simulink model "ps_model"  (R2025b)
settings: Solver=ode23tb  StartTime=0.0  StopTime=simlength  FixedStep=tc  MaxStep=tc
values from neighbouring files (symbols this model uses):
  omega_grid_emulator_nom = w_grid    (= 314.159265359)    [grid_emulator.m]
  omega_grid_nom = w_grid    (= 314.159265359)    [grid_emulator.m]
  ugrid_factor = 1    [grid_emulator.m]
  V_phase_normalization_factor = Vgrid_phase_normalization_factor    [grid_emulator.m]
  Vdc_base = 720    [grid_emulator.m]
  vn_eta_pu = 0    [grid_emulator.m]
  vn_xi_pu = 0    [grid_emulator.m]
  vp_xi_pu = 1    [grid_emulator.m]
undefined symbols (not defined in the file or in its folder): CFi, fnom, fPWM_INV, i_nom, ki_i, ki_u, kp_i, kp_u, Ld2_trafo_out, magnitude, n10, number_of_cells, omega_nom, Q, q1Kalman, q2Kalman, q3Kalman, R_RLload, Rd2_trafo_out, rKalman, tc, time_load_step, ts_afe, ts_inv, tsample, u_nom, Vdc_nom
libraries: fl_lib x120, nesl_utility x67, ee_lib x7, cstblocks x4, moving_average_filter x4, single_phase_transformer_lib x3, lithium_ion_cell_lib x1, simulink x1, threephase_inductor_lib x1
(part 3 of 4)

== system ps_model/inverter/MOS based inverter/inverter ==
  Simulink-PS Converter{,1..5} (6 alike) : nesl_utility/Simulink-PS Converter  PhysicalDomain=network_engine_domain  SubClassName=ps_input  LeftPortType=input  RightPortType=output  PseudoPeriodic=off  Frequencies=[]  NoiseDistribution=none  NoiseParameters=[]  Unit=V  AffineConversion=on  FilteringAndDerivatives=provide  SimscapeFilterOrder=1  InputFilterTimeConstant=0.001  UdotUserProvided=0
  mosfet_1 : Subsystem
      settings: PortSchema="{\"entries\":[{\"content\":{\"sides\":[{\"content\":{\"connectorIds\":[\"LConn1\"]},\"type\":\"ConnectorPlacement.EquallySpacedRectSide\",\"uuid\":\"9277da8d-d460-43e6-8478-dd662f15d226\"},{\"content\":{\"connectorIds\":[],\"side\":\"RIGHT\"},\"type\":\"ConnectorPlacement.EquallySpacedRectSide\",\"uuid\":\"a7ece396-f1d9-4f4f-a05b-db1fc65d6e1d\"},{\"content\":{\"connectorIds\":[\"LConn2\"],\"side\":\"TOP\"},\"type\":\"ConnectorPlacement.EquallySpacedRectSide\",\"uuid\":\"fdd70777-e9cf-4317-afb6-cae87f75d5b0\"},{\"content\":{\"connectorIds\":[\"RConn1\"],\"side\":\"BOTTOM\"},\"type\":\"ConnectorPlacement.EquallySpacedRectSide\",\"uuid\":\"2353ed68-b1a1-4775-9ca9-31e268d5443b\"}]},\"type\":\"ConnectorPlacement.EquallySpacedConnector\",\"uuid\":\"d5479f4c-4e65-4791-adcb-73df11f88590\"}],\"packageUris\":[\"http://schema.mathworks.com/mf0/Connector/R2020b\"],\"version\":\"1.0\"}"
  mosfet_2 : Subsystem
      settings: PortSchema="{\"entries\":[{\"content\":{\"sides\":[{\"content\":{\"connectorIds\":[\"LConn1\"]},\"type\":\"ConnectorPlacement.EquallySpacedRectSide\",\"uuid\":\"9277da8d-d460-43e6-8478-dd662f15d226\"},{\"content\":{\"connectorIds\":[],\"side\":\"RIGHT\"},\"type\":\"ConnectorPlacement.EquallySpacedRectSide\",\"uuid\":\"a7ece396-f1d9-4f4f-a05b-db1fc65d6e1d\"},{\"content\":{\"connectorIds\":[\"LConn2\"],\"side\":\"TOP\"},\"type\":\"ConnectorPlacement.EquallySpacedRectSide\",\"uuid\":\"fdd70777-e9cf-4317-afb6-cae87f75d5b0\"},{\"content\":{\"connectorIds\":[\"RConn1\"],\"side\":\"BOTTOM\"},\"type\":\"ConnectorPlacement.EquallySpacedRectSide\",\"uuid\":\"2353ed68-b1a1-4775-9ca9-31e268d5443b\"}]},\"type\":\"ConnectorPlacement.EquallySpacedConnector\",\"uuid\":\"d5479f4c-4e65-4791-adcb-73df11f88590\"}],\"packageUris\":[\"http://schema.mathworks.com/mf0/Connector/R2020b\"],\"version\":\"1.0\"}"
  mosfet_3 : Subsystem
      settings: PortSchema="{\"entries\":[{\"content\":{\"sides\":[{\"content\":{\"connectorIds\":[\"LConn1\"]},\"type\":\"ConnectorPlacement.EquallySpacedRectSide\",\"uuid\":\"9277da8d-d460-43e6-8478-dd662f15d226\"},{\"content\":{\"connectorIds\":[],\"side\":\"RIGHT\"},\"type\":\"ConnectorPlacement.EquallySpacedRectSide\",\"uuid\":\"a7ece396-f1d9-4f4f-a05b-db1fc65d6e1d\"},{\"content\":{\"connectorIds\":[\"LConn2\"],\"side\":\"TOP\"},\"type\":\"ConnectorPlacement.EquallySpacedRectSide\",\"uuid\":\"fdd70777-e9cf-4317-afb6-cae87f75d5b0\"},{\"content\":{\"connectorIds\":[\"RConn1\"],\"side\":\"BOTTOM\"},\"type\":\"ConnectorPlacement.EquallySpacedRectSide\",\"uuid\":\"2353ed68-b1a1-4775-9ca9-31e268d5443b\"}]},\"type\":\"ConnectorPlacement.EquallySpacedConnector\",\"uuid\":\"d5479f4c-4e65-4791-adcb-73df11f88590\"}],\"packageUris\":[\"http://schema.mathworks.com/mf0/Connector/R2020b\"],\"version\":\"1.0\"}"
  mosfet_4 : Subsystem
      settings: PortSchema="{\"entries\":[{\"content\":{\"sides\":[{\"content\":{\"connectorIds\":[\"LConn1\"]},\"type\":\"ConnectorPlacement.EquallySpacedRectSide\",\"uuid\":\"9277da8d-d460-43e6-8478-dd662f15d226\"},{\"content\":{\"connectorIds\":[],\"side\":\"RIGHT\"},\"type\":\"ConnectorPlacement.EquallySpacedRectSide\",\"uuid\":\"a7ece396-f1d9-4f4f-a05b-db1fc65d6e1d\"},{\"content\":{\"connectorIds\":[\"LConn2\"],\"side\":\"TOP\"},\"type\":\"ConnectorPlacement.EquallySpacedRectSide\",\"uuid\":\"fdd70777-e9cf-4317-afb6-cae87f75d5b0\"},{\"content\":{\"connectorIds\":[\"RConn1\"],\"side\":\"BOTTOM\"},\"type\":\"ConnectorPlacement.EquallySpacedRectSide\",\"uuid\":\"2353ed68-b1a1-4775-9ca9-31e268d5443b\"}]},\"type\":\"ConnectorPlacement.EquallySpacedConnector\",\"uuid\":\"d5479f4c-4e65-4791-adcb-73df11f88590\"}],\"packageUris\":[\"http://schema.mathworks.com/mf0/Connector/R2020b\"],\"version\":\"1.0\"}"
  mosfet_5 : Subsystem
      settings: PortSchema="{\"entries\":[{\"content\":{\"sides\":[{\"content\":{\"connectorIds\":[\"LConn1\"]},\"type\":\"ConnectorPlacement.EquallySpacedRectSide\",\"uuid\":\"9277da8d-d460-43e6-8478-dd662f15d226\"},{\"content\":{\"connectorIds\":[],\"side\":\"RIGHT\"},\"type\":\"ConnectorPlacement.EquallySpacedRectSide\",\"uuid\":\"a7ece396-f1d9-4f4f-a05b-db1fc65d6e1d\"},{\"content\":{\"connectorIds\":[\"LConn2\"],\"side\":\"TOP\"},\"type\":\"ConnectorPlacement.EquallySpacedRectSide\",\"uuid\":\"fdd70777-e9cf-4317-afb6-cae87f75d5b0\"},{\"content\":{\"connectorIds\":[\"RConn1\"],\"side\":\"BOTTOM\"},\"type\":\"ConnectorPlacement.EquallySpacedRectSide\",\"uuid\":\"2353ed68-b1a1-4775-9ca9-31e268d5443b\"}]},\"type\":\"ConnectorPlacement.EquallySpacedConnector\",\"uuid\":\"d5479f4c-4e65-4791-adcb-73df11f88590\"}],\"packageUris\":[\"http://schema.mathworks.com/mf0/Connector/R2020b\"],\"version\":\"1.0\"}"
  mosfet_6 : Subsystem
      settings: PortSchema="{\"entries\":[{\"content\":{\"sides\":[{\"content\":{\"connectorIds\":[\"LConn1\"]},\"type\":\"ConnectorPlacement.EquallySpacedRectSide\",\"uuid\":\"9277da8d-d460-43e6-8478-dd662f15d226\"},{\"content\":{\"connectorIds\":[],\"side\":\"RIGHT\"},\"type\":\"ConnectorPlacement.EquallySpacedRectSide\",\"uuid\":\"a7ece396-f1d9-4f4f-a05b-db1fc65d6e1d\"},{\"content\":{\"connectorIds\":[\"LConn2\"],\"side\":\"TOP\"},\"type\":\"ConnectorPlacement.EquallySpacedRectSide\",\"uuid\":\"fdd70777-e9cf-4317-afb6-cae87f75d5b0\"},{\"content\":{\"connectorIds\":[\"RConn1\"],\"side\":\"BOTTOM\"},\"type\":\"ConnectorPlacement.EquallySpacedRectSide\",\"uuid\":\"2353ed68-b1a1-4775-9ca9-31e268d5443b\"}]},\"type\":\"ConnectorPlacement.EquallySpacedConnector\",\"uuid\":\"d5479f4c-4e65-4791-adcb-73df11f88590\"}],\"packageUris\":[\"http://schema.mathworks.com/mf0/Connector/R2020b\"],\"version\":\"1.0\"}"
  udc(+) : PMIOPort  Side=Left
  udc(-) : PMIOPort  Port=2  Side=Left
  u : PMIOPort  Port=3  Side=Right
  v : PMIOPort  Port=4  Side=Right
  w : PMIOPort  Port=5  Side=Right
  wires:
  [gm6] -> Simulink-PS Converter5/1
  [gm2] -> Simulink-PS Converter1/1
  [gm3] -> Simulink-PS Converter2/1
  [gm4] -> Simulink-PS Converter3/1
  [gm5] -> Simulink-PS Converter4/1
  [gm1] -> Simulink-PS Converter/1
  connections:
  mosfet_6/LConn2 -- mosfet_5/RConn1 -- w/RConn1
  mosfet_1/RConn1 -- u/RConn1 -- mosfet_2/LConn2
  mosfet_5/LConn2 -- udc(+)/RConn1 -- mosfet_1/LConn2 -- mosfet_3/LConn2
  mosfet_4/LConn2 -- mosfet_3/RConn1 -- v/RConn1
  mosfet_6/RConn1 -- udc(-)/RConn1 -- mosfet_2/RConn1 -- mosfet_4/RConn1
  mosfet_1/LConn1 -- Simulink-PS Converter/RConn1
  mosfet_2/LConn1 -- Simulink-PS Converter1/RConn1
  mosfet_4/LConn1 -- Simulink-PS Converter3/RConn1
  mosfet_6/LConn1 -- Simulink-PS Converter5/RConn1
  mosfet_3/LConn1 -- Simulink-PS Converter2/RConn1
  mosfet_5/LConn1 -- Simulink-PS Converter4/RConn1

== system ps_model/inverter/MOS based inverter/spwm ==
  ab : Inport
  enable : Inport  Port=2
  pwm_phase : Inport  Port=3
  -1<x<1 : Saturate  UpperLimit=1  LowerLimit=-1
  Data Type Conversion1 : DataTypeConversion  OutDataTypeStr=double  SaturateOnIntegerOverflow=off  RndMeth=Floor
  Data Type Conversion2 : DataTypeConversion  OutDataTypeStr=double  SaturateOnIntegerOverflow=off  RndMeth=Floor
  Data Type Conversion3 : DataTypeConversion  OutDataTypeStr=double  SaturateOnIntegerOverflow=off  RndMeth=Floor
  Demux : Demux  Outputs=2
  conditioning : MATLAB Function  TreatAsAtomicUnit=on  SystemSampleTime=ts_inv
  modulator1 : Subsystem
  uvw2alphabeta : MATLAB Function  TreatAsAtomicUnit=on  SystemSampleTime=ts_inv
  cmd_gates : Outport
  wires:
  -1<x<1/1 -> Demux/1
  modulator1/1(cmd_gates) -> cmd_gates/1
  pwm_phase/1 -> modulator1/4(phase)
  Data Type Conversion1/1 -> modulator1/1(u)  "du"
  Data Type Conversion2/1 -> modulator1/2(v)  "dv"
  Data Type Conversion3/1 -> modulator1/3(w)  "dw"
  ab/1 -> -1<x<1/1
  Demux/1 -> uvw2alphabeta/1(alpha)
  Demux/2 -> uvw2alphabeta/2(beta)
  uvw2alphabeta/1(u) -> conditioning/1(u1)  "mu"
  uvw2alphabeta/2(v) -> conditioning/2(v1)  "mv"
  uvw2alphabeta/3(w) -> conditioning/3(w1)  "mw"
  conditioning/1(u2) -> Data Type Conversion1/1  "mu"
  conditioning/2(v2) -> Data Type Conversion2/1  "mv"
  conditioning/3(w2) -> Data Type Conversion3/1  "mw"

== system ps_model/inverter/MOS based inverter/sv_pwm ==
  ab : Inport
  enable : Inport  Port=2
  pwm_phase : Inport  Port=3
  -1<x<1 : Saturate  UpperLimit=1  LowerLimit=-1
  Bus Selector : BusSelector  OutputSignals=da,db,dc
  C Caller : CCaller  FunctionName=sv_pwm_process_simulink  PortSpecificationStruct="%)30     .    V @   8    (     @         %    \"     4    !     0         %  0 \"0    $    _    07)G3F%M90  4&]R=$YA;64 4V-O<&4     26YD97@     5'EP90      4VEZ90      27-';&]B86P   X    P    !@    @    $          4    (     0    ,    !         !   P!O=70 #@   #     &    \"     0         !0    @    !     P    $         $  # &]U=  .    .     8    (    !          %    \"     $    &     0         0   ...(+2669 chars)"  SampleTime=ts_inv
  Constant : Constant  Value=ts_inv
  Data Type Conversion1 : DataTypeConversion  OutDataTypeStr=double  SaturateOnIntegerOverflow=off  RndMeth=Floor
  Data Type Conversion15 : DataTypeConversion  OutDataTypeStr=single  SaturateOnIntegerOverflow=off  RndMeth=Floor
  Data Type Conversion16 : DataTypeConversion  OutDataTypeStr=single  SaturateOnIntegerOverflow=off  RndMeth=Floor
  Data Type Conversion17 : DataTypeConversion  OutDataTypeStr=uint32  SaturateOnIntegerOverflow=off  RndMeth=Floor
  Data Type Conversion18 : DataTypeConversion  OutDataTypeStr=single  SaturateOnIntegerOverflow=off  RndMeth=Floor
  Data Type Conversion2 : DataTypeConversion  OutDataTypeStr=double  SaturateOnIntegerOverflow=off  RndMeth=Floor
  Data Type Conversion3 : DataTypeConversion  OutDataTypeStr=double  SaturateOnIntegerOverflow=off  RndMeth=Floor
  Demux : Demux  Outputs=2
  Gain : Gain  Gain=sqrt(3)/2
  Zero-Order Hold{,1..3} (4 alike) : ZeroOrderHold  SampleTime=ts_inv
  modulator1 : Subsystem
  cmd_gates : Outport
  wires:
  Demux/2 -> Data Type Conversion15/1
  ab/1 -> -1<x<1/1
  Data Type Conversion3/1 -> modulator1/3(w)  "dw"
  C Caller/1 -> Bus Selector/1  "out"
  Data Type Conversion15/1 -> Zero-Order Hold1/1
  Zero-Order Hold3/1 -> C Caller/4
  Data Type Conversion17/1 -> Zero-Order Hold3/1
  Zero-Order Hold1/1 -> C Caller/2
  Data Type Conversion16/1 -> Zero-Order Hold2/1
  Data Type Conversion2/1 -> modulator1/2(v)  "dv"
  enable/1 -> Data Type Conversion17/1
  Data Type Conversion18/1 -> Zero-Order Hold/1
  Constant/1 -> Data Type Conversion16/1
  Zero-Order Hold2/1 -> C Caller/3
  Zero-Order Hold/1 -> C Caller/1
  Data Type Conversion1/1 -> modulator1/1(u)  "du"
  Demux/1 -> Data Type Conversion18/1
  pwm_phase/1 -> modulator1/4(phase)
  modulator1/1(cmd_gates) -> cmd_gates/1
  -1<x<1/1 -> Gain/1
  Gain/1 -> Demux/1
  Bus Selector/3 -> Data Type Conversion3/1  "<dc>"
  Bus Selector/2 -> Data Type Conversion2/1  "<db>"
  Bus Selector/1 -> Data Type Conversion1/1  "<da>"

== system ps_model/inverter/instantaneus_power/abc2alphabeta ==
  a : Inport
  b : Inport  Port=2
  c : Inport  Port=3
  abc2alphabeta : Subsystem
  vline_alpha : Outport  VectorParamsAs1DForOutWhenUnconnected=off
  vline_beta : Outport  Port=2  VectorParamsAs1DForOutWhenUnconnected=off
  wires:
  a/1 -> abc2alphabeta/1(a)
  b/1 -> abc2alphabeta/2(b)
  c/1 -> abc2alphabeta/3(c)
  abc2alphabeta/2("beta ") -> vline_beta/1
  abc2alphabeta/1("alpha ") -> vline_alpha/1

== system ps_model/inverter/instantaneus_power/abc2alphabeta  ==
  a : Inport
  b : Inport  Port=2
  c : Inport  Port=3
  abc->alphabeta : Subsystem
  i_line_alpha : Outport  VectorParamsAs1DForOutWhenUnconnected=off
  i_line_beta : Outport  Port=2  VectorParamsAs1DForOutWhenUnconnected=off
  wires:
  abc->alphabeta/1("alpha ") -> i_line_alpha/1
  abc->alphabeta/2("beta ") -> i_line_beta/1
  c/1 -> abc->alphabeta/3(c)
  b/1 -> abc->alphabeta/2(b)
  a/1 -> abc->alphabeta/1(a)

== system ps_model/inverter/instantaneus_power/moving_avarage1 ==
  In : Inport
  Constant : Constant  Value=omega_nom
  Zero-Order Hold : ZeroOrderHold  SampleTime=ts_inv
  dmavg_flt : moving_average_filter/dmavg_flt  ts=ts_inv  enable_time=0.025
  Mean : Outport  VectorParamsAs1DForOutWhenUnconnected=off
  wires:
  Constant/1 -> dmavg_flt/2
  dmavg_flt/1 -> Mean/1
  In/1 -> Zero-Order Hold/1
  Zero-Order Hold/1 -> dmavg_flt/1

== system ps_model/inverter/instantaneus_power/moving_avarage2 ==
  In : Inport
  Constant : Constant  Value=omega_nom
  Zero-Order Hold : ZeroOrderHold  SampleTime=ts_inv
  dmavg_flt : moving_average_filter/dmavg_flt  ts=ts_inv  enable_time=0.025
  Mean : Outport  VectorParamsAs1DForOutWhenUnconnected=off
  wires:
  Zero-Order Hold/1 -> dmavg_flt/1
  In/1 -> Zero-Order Hold/1
  dmavg_flt/1 -> Mean/1
  Constant/1 -> dmavg_flt/2

== system ps_model/inverter/instantaneus_power/rms ==
  In1 : Inport
  Gain : Gain  Gain=n10-1
  Gain1 : Gain  Gain=1/n10
  Math Function : Math  Operator=magnitude^2  SignedPower=on
  Sqrt : Sqrt
  Sum : Sum  Inputs=|++
  Unit Delay : UnitDelay  SampleTime=ts_afe  HasFrameUpgradeWarning=on
  Out1 : Outport  VectorParamsAs1DForOutWhenUnconnected=off
  wires:
  In1/1 -> Math Function/1
  Sum/1 -> Gain1/1
  Gain1/1 -> Sqrt/1, Unit Delay/1
  Unit Delay/1 -> Gain/1
  Math Function/1 -> Sum/1
  Sqrt/1 -> Out1/1
  Gain/1 -> Sum/2

== system ps_model/inverter/instantaneus_power/rms1 ==
  In1 : Inport
  Gain : Gain  Gain=n10-1
  Gain1 : Gain  Gain=1/n10
  Math Function : Math  Operator=magnitude^2  SignedPower=on
  Sqrt : Sqrt
  Sum : Sum  Inputs=|++
  Unit Delay : UnitDelay  SampleTime=ts_afe  HasFrameUpgradeWarning=on
  Out1 : Outport  VectorParamsAs1DForOutWhenUnconnected=off
  wires:
  Gain/1 -> Sum/2
  Sqrt/1 -> Out1/1
  Math Function/1 -> Sum/1
  Unit Delay/1 -> Gain/1
  Gain1/1 -> Unit Delay/1, Sqrt/1
  Sum/1 -> Gain1/1
  In1/1 -> Math Function/1

== system ps_model/inverter/instantaneus_power/rms2 ==
  In1 : Inport
  Gain : Gain  Gain=n10-1
  Gain1 : Gain  Gain=1/n10
  Math Function : Math  Operator=magnitude^2  SignedPower=on
  Sqrt : Sqrt
  Sum : Sum  Inputs=|++
  Unit Delay : UnitDelay  SampleTime=ts_afe  HasFrameUpgradeWarning=on
  Out1 : Outport  VectorParamsAs1DForOutWhenUnconnected=off
  wires:
  In1/1 -> Math Function/1
  Sum/1 -> Gain1/1
  Gain1/1 -> Sqrt/1, Unit Delay/1
  Unit Delay/1 -> Gain/1
  Math Function/1 -> Sum/1
  Sqrt/1 -> Out1/1
  Gain/1 -> Sum/2

== system ps_model/inverter/instantaneus_power/rms3 ==
  In1 : Inport
  Gain : Gain  Gain=n10-1
  Gain1 : Gain  Gain=1/n10
  Math Function : Math  Operator=magnitude^2  SignedPower=on
  Sqrt : Sqrt
  Sum : Sum  Inputs=|++
  Unit Delay : UnitDelay  SampleTime=ts_afe  HasFrameUpgradeWarning=on
  Out1 : Outport  VectorParamsAs1DForOutWhenUnconnected=off
  wires:
  Gain/1 -> Sum/2
  Sqrt/1 -> Out1/1
  Math Function/1 -> Sum/1
  Unit Delay/1 -> Gain/1
  Gain1/1 -> Unit Delay/1, Sqrt/1
  Sum/1 -> Gain1/1
  In1/1 -> Math Function/1

== system ps_model/inverter/instantaneus_power/rms4 ==
  In1 : Inport
  Gain : Gain  Gain=n10-1
  Gain1 : Gain  Gain=1/n10
  Math Function : Math  Operator=magnitude^2  SignedPower=on
  Sqrt : Sqrt
  Sum : Sum  Inputs=|++
  Unit Delay : UnitDelay  SampleTime=ts_afe  HasFrameUpgradeWarning=on
  Out1 : Outport  VectorParamsAs1DForOutWhenUnconnected=off
  wires:
  In1/1 -> Math Function/1
  Sum/1 -> Gain1/1
  Gain1/1 -> Sqrt/1, Unit Delay/1
  Unit Delay/1 -> Gain/1
  Math Function/1 -> Sum/1
  Sqrt/1 -> Out1/1
  Gain/1 -> Sum/2

== system ps_model/inverter/instantaneus_power/rms5 ==
  In1 : Inport
  Gain : Gain  Gain=n10-1
  Gain1 : Gain  Gain=1/n10
  Math Function : Math  Operator=magnitude^2  SignedPower=on
  Sqrt : Sqrt
  Sum : Sum  Inputs=|++
  Unit Delay : UnitDelay  SampleTime=ts_afe  HasFrameUpgradeWarning=on
  Out1 : Outport  VectorParamsAs1DForOutWhenUnconnected=off
  wires:
  Gain/1 -> Sum/2
  Sqrt/1 -> Out1/1
  Math Function/1 -> Sum/1
  Unit Delay/1 -> Gain/1
  Gain1/1 -> Unit Delay/1, Sqrt/1
  Sum/1 -> Gain1/1
  In1/1 -> Math Function/1

== system ps_model/rectifier/rectifier/dclink_measure ==
  Controlled Voltage Source : fl_lib/Electrical/Electrical Sources/Controlled Voltage Source
  Current Sensor1 : fl_lib/Electrical/Electrical Sensors/Current Sensor
  Electrical Reference : fl_lib/Electrical/Electrical Elements/Electrical Reference
  Gain : Gain  Gain=107.4e3
  Gain1 : Gain  Gain=1/Vdc_base
  Quantizer : Quantizer  QuantizationInterval=VoltageQuantization
  R_derating : Subsystem  Commented=on
  Resistor : fl_lib/Electrical/Electrical Elements/Resistor  R=107.4 kOhm  i_specify=off  i_priority=None  i=0 A  i_nominal_specify=off  i_nominal_value=1  i_nominal_unit=A  v_specify=off  v_priority=None  v=0 V  v_nominal_specify=off  v_nominal_value=1  v_nominal_unit=V
  Saturation : Saturate  UpperLimit=inf  LowerLimit=1
  Simulink-PS Converter : nesl_utility/Simulink-PS Converter  PhysicalDomain=network_engine_domain  SubClassName=ps_input  LeftPortType=input  RightPortType=output  PseudoPeriodic=off  Frequencies=[]  NoiseDistribution=none  NoiseParameters=[]  Unit=Ohm  AffineConversion=off  FilteringAndDerivatives=provide  SimscapeFilterOrder=1  InputFilterTimeConstant=0.001  UdotUserProvided=0
  Variable Resistor : fl_lib/Electrical/Electrical Elements/Variable Resistor  Rmin=0 Ohm  thermalEnable=false  thermal_mass=1 J/K  i_specify=off  i_priority=None  i=0 A  i_nominal_specify=off  i_nominal_value=1  i_nominal_unit=A  v_specify=off  v_priority=None  v=0 V  v_nominal_specify=off  v_nominal_value=1  v_nominal_unit=V  T_specify=off  T_priority=None  T=300 K  T_nominal_specify=off  T_nominal_value=1  T_nominal_unit=K
  dclink_voltage_measure_comparison_mod1 : Scope  NumInputPorts=3
      settings: SampleTime=tc  ActiveDisplayYMinimum=455.76686  ActiveDisplayYMaximum=735.66715
  im_udc : nesl_utility/PS-Simulink Converter  PhysicalDomain=network_engine_domain  SubClassName=ps_output  LeftPortType=input  RightPortType=output  PseudoPeriodic=off  Frequencies=[]  VectorFormat=1-D array  Unit=A  AffineConversion=on
  udc : PMIOPort  Side=Left
  tag scope: vdc_pu_mod1=global
  wires:
  Gain/1 -> Saturation/1, dclink_voltage_measure_comparison_mod1/1  "measure_si"
  Quantizer/1 -> Gain1/1
  Saturation/1 -> Quantizer/1
  im_udc/1 -> Gain/1
  Gain1/1 -> dclink_voltage_measure_comparison_mod1/2, [vdc_pu_mod1]  "measure_pu"
  [udc_mod1] -> dclink_voltage_measure_comparison_mod1/3  "real"
  R_derating/1(DR) -> Simulink-PS Converter/1
  connections:
  udc/RConn1 -- Controlled Voltage Source/RConn1
  Resistor/RConn1 -- Variable Resistor/LConn2
  Current Sensor1/RConn1 -- im_udc/LConn1
  Current Sensor1/RConn2 -- Electrical Reference/LConn1 -- Controlled Voltage Source/RConn2
  Current Sensor1/LConn1 -- Variable Resistor/RConn1
  Simulink-PS Converter/RConn1 -- Variable Resistor/LConn1
  Controlled Voltage Source/LConn1 -- Resistor/LConn1

== system ps_model/battery_system/battery_system/LithiumIonBattery/SOC_estimator ==
  Kalman_observer : Subsystem
  SOC*/SOC : Scope  Commented=on  NumInputPorts=2
      settings: SampleTime=tsample  ActiveDisplayYMinimum=-0.16149  ActiveDisplayYMaximum=0.90685
  Selector1 : Selector  InputPortWidth=3  IndexOptions=Index vector (dialog)  Indices=3  OutputSizes=1
  h_hat/h : Scope  Commented=on  NumInputPorts=2
      settings: SampleTime=tsample  ActiveDisplayYMinimum=-0.13002  ActiveDisplayYMaximum=0.15534  DataLoggingVariableName=ScopeData2
  i_out/v_out : Scope  Commented=on  NumInputPorts=2
      settings: SampleTime=tsample  ActiveDisplayYMinimum=-467.64425  ActiveDisplayYMaximum=280.87629  DataLoggingVariableName=ScopeData3
  soc/iout : Scope  Commented=on  NumInputPorts=2
      settings: SampleTime=tsample  ActiveDisplayYMinimum=0.19925  ActiveDisplayYMaximum=0.20008  DataLoggingVariableName=ScopeData4
  wires:
  Kalman_observer/2(SOC) -> SOC*/SOC/2
  Kalman_observer/1(x(k+1|k)) -> Selector1/1
  [im] -> i_out/v_out/1  "im+noise"
  [h] -> h_hat/h/2
  [SOC] -> soc/iout/1, SOC*/SOC/1
  Selector1/1 -> h_hat/h/1  "h_hat(z)"
  [vout] -> Kalman_observer/1(vout(k)), i_out/v_out/2
  [icell] -> soc/iout/2

== system ps_model/battery_system/battery_system/LithiumIonBattery/lithium ion cell analytical ocv ==
  Current Sensor : fl_lib/Electrical/Electrical Sensors/Current Sensor
  Electrical Reference : fl_lib/Electrical/Electrical Elements/Electrical Reference
  PS Constant : fl_lib/Physical Signals/Sources/PS Constant  constant=298.15 K
  PS-Simulink Converter{,1..4} (5 alike) : nesl_utility/PS-Simulink Converter  PhysicalDomain=network_engine_domain  SubClassName=ps_output  LeftPortType=input  RightPortType=output  PseudoPeriodic=off  Frequencies=[]  VectorFormat=1-D array  Unit=inherit  AffineConversion=off
  Voltage Sensor : fl_lib/Electrical/Electrical Sensors/Voltage Sensor
  lithium-ion battery with analytical OCV : lithium_ion_cell_lib/lithium-ion Cell with analytical OCV  Qcell=Q hr*A  N=number_of_cells  E_1=E1 V  E0=E0 V  E1=E1 V  E2=E2 V  E3=E3 V  Elog=Elog V  R0=R0 Ohm  R1=R1 Ohm  C1=C1 F  M=M V  alpha=alpha  u_specify=off  u_priority=High  u=Vdc V  u_nominal_specify=off  u_nominal_unit=V  u_nominal_value=1  u_ocv_specify=off  u_ocv_priority=High  u_ocv=Vdc V  u_ocv_nominal_specify=off  u_ocv_nominal_unit=V  u_ocv_nominal_value=1  icell_specify=off  icell_priority=None  icell=0 A  icell_nominal_specify=off  icell_nominal_unit=A  icell_nominal_value=1  i_r1_specify=off  i_r1_priority=None  i_r1=0 A  i_r1_nominal_specify=off  i_r1_nominal_unit=A  i_r1_nominal_value=1  z_specify=on  z_priority=High  z=soc_init  z_nominal_specify=off  z_nominal_unit=1  z_nominal_value=1  h_specify=off  h_priority=High  h=0  h_nominal_specify=off  h_nominal_unit=1  h_nominal_value=1
      settings: InternalSimscapePortConfiguration="{\"Bottom\":[],\"Left\":[{\"id\":\"T\",\"label\":\"T\",\"type\":\"input\"}],\"Right\":[{\"id\":\"u_p\",\"label\":\"u+\",\"type\":\"foundation.electrical.electrical\"},{\"id\":\"u_n\",\"label\":\"u-\",\"type\":\"foundation.electrical.electrical\"},{\"id\":\"z_out\",\"label\":\"SOC\",\"type\":\"output\"},{\"id\":\"i_r1_out\",\"label\":\"i_r1\",\"type\":\"output\"},{\"id\":\"h_out\",\"label\":\"hysteresis\",\"type\":\"output\"}],\"Top\":[]}"
  white_noise : Subsystem
  U+ : PMIOPort  Side=Right
  U- : PMIOPort  Port=2  Side=Right
  tag scope: SOC=global, h=global, icell=global, im=global, vout=global
  wires:
  PS-Simulink Converter/1 -> [vout]  "vout(k)"
  PS-Simulink Converter1/1 -> white_noise/1(in)  "i(k)"
  white_noise/1(out) -> [im]
  PS-Simulink Converter4/1 -> [h]  "h(t)"
  PS-Simulink Converter2/1 -> [icell]  "icell"
  PS-Simulink Converter3/1 -> [SOC]  "SOC*"
  connections:
  lithium-ion battery with analytical OCV/LConn1 -- PS Constant/RConn1
  PS-Simulink Converter/LConn1 -- Voltage Sensor/RConn1
  Current Sensor/RConn2 -- Voltage Sensor/LConn1 -- U+/RConn1
  Electrical Reference/LConn1 -- Voltage Sensor/RConn2 -- U-/RConn1 -- lithium-ion battery with analytical OCV/RConn2
  Current Sensor/RConn1 -- PS-Simulink Converter1/LConn1
  lithium-ion battery with analytical OCV/RConn1 -- Current Sensor/LConn1
  lithium-ion battery with analytical OCV/RConn3 -- PS-Simulink Converter3/LConn1
  lithium-ion battery with analytical OCV/RConn4 -- PS-Simulink Converter2/LConn1
  lithium-ion battery with analytical OCV/RConn5 -- PS-Simulink Converter4/LConn1

== system ps_model/grid/grid_emulator/grid_emulator/phase_gen ==
  Constant4 : Constant  Value=omega_grid_emulator_nom
  Integrator : Integrator
  bounder1 : MATLAB Function  TreatAsAtomicUnit=on
  grid_emu_phase : Outport  VectorParamsAs1DForOutWhenUnconnected=off
  tag scope: gamma_grid_emulator=global
  wires:
  bounder1/1(y) -> [gamma_grid_emulator], grid_emu_phase/1  "grid_emu_phase"
  Constant4/1 -> Integrator/1
  Integrator/1 -> bounder1/1(u)

== system ps_model/grid/grid_emulator/grid_emulator/voltage_reference ==
  grid_emu_phase : Inport
  Vxi_p : Inport  Port=2
  Vxi_n : Inport  Port=3
  Veta_n : Inport  Port=4
  Constant2 : Constant  Value=0
  Sum1 : Sum  Inputs=|++
  Sum4 : Sum  Inputs=|++
  alphabeta2abc : MATLAB Function  TreatAsAtomicUnit=on
  xieta2alphabeta_neg : MATLAB Function  TreatAsAtomicUnit=on
  xieta2alphabeta_pos : MATLAB Function  TreatAsAtomicUnit=on
  V1_ref : Outport  VectorParamsAs1DForOutWhenUnconnected=off
  V2_ref : Outport  Port=2  VectorParamsAs1DForOutWhenUnconnected=off
  V3_ref : Outport  Port=3  VectorParamsAs1DForOutWhenUnconnected=off
  wires:
  xieta2alphabeta_pos/1(alpha) -> Sum1/1
  Sum1/1 -> alphabeta2abc/1(alpha)
  xieta2alphabeta_pos/2(beta) -> Sum4/1
  Sum4/1 -> alphabeta2abc/2(beta)
  xieta2alphabeta_neg/1(alpha) -> Sum1/2
  xieta2alphabeta_neg/2(beta) -> Sum4/2
  grid_emu_phase/1 -> xieta2alphabeta_neg/3(gamma), xieta2alphabeta_pos/3(gamma)
  Vxi_p/1 -> xieta2alphabeta_pos/1(xi)
  Constant2/1 -> xieta2alphabeta_pos/2(eta)
  Vxi_n/1 -> xieta2alphabeta_neg/1(xi)
  Veta_n/1 -> xieta2alphabeta_neg/2(eta)
  alphabeta2abc/1(a) -> V1_ref/1
  alphabeta2abc/2(b) -> V2_ref/1
  alphabeta2abc/3(c) -> V3_ref/1

== system ps_model/grid/grid_emulator/grid_emulator/voltage_source ==
  Constant : Constant  Value=vp_xi_pu
  Constant1 : Constant  Value=vn_xi_pu
  Constant2 : Constant  Value=vn_eta_pu
  Gain1 : Gain  Gain=V_phase_normalization_factor
  Gain2 : Gain  Gain=ugrid_factor
  Gain3 : Gain  Gain=ugrid_factor
  Gain4 : Gain  Gain=ugrid_factor
  Gain7 : Gain  Gain=V_phase_normalization_factor
  Gain8 : Gain  Gain=V_phase_normalization_factor
  LTI System3 : cstblocks/LTI System  sys=LVRT_flt_ss_c  IC=[]  PadeOrder=0
  LTI System4 : cstblocks/LTI System  sys=LVRT_flt_ss_c  IC=[]  PadeOrder=0
  LTI System5 : cstblocks/LTI System  sys=LVRT_flt_ss_c  IC=[]  PadeOrder=0
  vp_xi : Outport  VectorParamsAs1DForOutWhenUnconnected=off
  vn_xi : Outport  Port=2  VectorParamsAs1DForOutWhenUnconnected=off
  vn_eta : Outport  Port=3  VectorParamsAs1DForOutWhenUnconnected=off
  wires:
  LTI System3/1 -> Gain7/1
  LTI System4/1 -> Gain8/1
  Gain7/1 -> Gain2/1
  Gain8/1 -> Gain3/1
  Gain1/1 -> Gain4/1
  LTI System5/1 -> Gain1/1
  Gain2/1 -> vp_xi/1
  Gain3/1 -> vn_xi/1
  Gain4/1 -> vn_eta/1
  Constant2/1 -> LTI System5/1
  Constant1/1 -> LTI System4/1
  Constant/1 -> LTI System3/1

== system ps_model/grid/instantaneus_power/abc2alphabeta/abc2alphabeta ==
  a : Inport
  b : Inport  Port=2
  c : Inport  Port=3
  Gain1 : Gain  Gain=-1/2
  Gain11 : Gain  Gain=-1/2
  Gain2 : Gain  Gain=0
  Gain3 : Gain  Gain=sqrt(3)/2
  Gain4 : Gain  Gain=-sqrt(3)/2
  Gain8 : Gain  Gain=2/3
  Gain9 : Gain  Gain=2/3
  Sum : Sum  Inputs=+++
  Sum1 : Sum  Inputs=+++
  "alpha " : Outport  VectorParamsAs1DForOutWhenUnconnected=off
  "beta " : Outport  Port=2  VectorParamsAs1DForOutWhenUnconnected=off
  wires:
  Gain11/1 -> Sum/2
  Gain1/1 -> Sum/3
  Gain9/1 -> "beta "/1
  Gain8/1 -> "alpha "/1
  Gain2/1 -> Sum1/1
  Gain3/1 -> Sum1/2
  Gain4/1 -> Sum1/3
  a/1 -> Gain2/1, Sum/1
  c/1 -> Gain4/1, Gain1/1
  b/1 -> Gain3/1, Gain11/1
  Sum/1 -> Gain8/1
  Sum1/1 -> Gain9/1

== system ps_model/grid/instantaneus_power/abc2alphabeta /abc->alphabeta ==
  a : Inport
  b : Inport  Port=2
  c : Inport  Port=3
  Gain1 : Gain  Gain=-1/2
  Gain11 : Gain  Gain=-1/2
  Gain2 : Gain  Gain=0
  Gain3 : Gain  Gain=sqrt(3)/2
  Gain4 : Gain  Gain=-sqrt(3)/2
  Gain8 : Gain  Gain=2/3
  Gain9 : Gain  Gain=2/3
  Sum : Sum  Inputs=+++
  Sum1 : Sum  Inputs=+++
  "alpha " : Outport  VectorParamsAs1DForOutWhenUnconnected=off
  "beta " : Outport  Port=2  VectorParamsAs1DForOutWhenUnconnected=off
  wires:
  Sum1/1 -> Gain9/1
  Sum/1 -> Gain8/1
  b/1 -> Gain11/1, Gain3/1
  c/1 -> Gain1/1, Gain4/1
  a/1 -> Sum/1, Gain2/1
  Gain4/1 -> Sum1/3
  Gain3/1 -> Sum1/2
  Gain2/1 -> Sum1/1
  Gain8/1 -> "alpha "/1
  Gain9/1 -> "beta "/1
  Gain1/1 -> Sum/3
  Gain11/1 -> Sum/2

== system ps_model/inverter/MOS based inverter/inverter/mosfet_1 ==
  Diode : fl_lib/Electrical/Electrical Elements/Diode  Vf=Vgamma V  Ron=Ron Ohm  Goff=1e-8 1/Ohm  i_specify=off  i_priority=None  i=0 A  i_nominal_specify=off  i_nominal_value=1  i_nominal_unit=A  v_specify=off  v_priority=None  v=0 V  v_nominal_specify=off  v_nominal_value=1  v_nominal_unit=V
  Switch : fl_lib/Electrical/Electrical Elements/Switch  R_closed=Ron Ohm  G_open=1e-8 1/Ohm  Threshold=7.5  i_specify=off  i_priority=None  i=0 A  i_nominal_specify=off  i_nominal_value=1  i_nominal_unit=A  v_specify=off  v_priority=None  v=0 V  v_nominal_specify=off  v_nominal_value=1  v_nominal_unit=V
  G : PMIOPort  Side=Left
  C : PMIOPort  Port=2  Side=Left
  E : PMIOPort  Port=3  Side=Right
  connections:
  Diode/LConn1 -- E/RConn1 -- Switch/LConn1
  Switch/RConn1 -- G/RConn1
  Diode/RConn1 -- C/RConn1 -- Switch/RConn2

== system ps_model/inverter/MOS based inverter/inverter/mosfet_2 ==
  Diode : fl_lib/Electrical/Electrical Elements/Diode  Vf=Vgamma V  Ron=Ron Ohm  Goff=1e-8 1/Ohm  i_specify=off  i_priority=None  i=0 A  i_nominal_specify=off  i_nominal_value=1  i_nominal_unit=A  v_specify=off  v_priority=None  v=0 V  v_nominal_specify=off  v_nominal_value=1  v_nominal_unit=V
  Switch : fl_lib/Electrical/Electrical Elements/Switch  R_closed=Ron Ohm  G_open=1e-8 1/Ohm  Threshold=7.5  i_specify=off  i_priority=None  i=0 A  i_nominal_specify=off  i_nominal_value=1  i_nominal_unit=A  v_specify=off  v_priority=None  v=0 V  v_nominal_specify=off  v_nominal_value=1  v_nominal_unit=V
  G : PMIOPort  Side=Left
  C : PMIOPort  Port=2  Side=Left
  E : PMIOPort  Port=3  Side=Right
  connections:
  Switch/RConn2 -- C/RConn1 -- Diode/RConn1
  Switch/RConn1 -- G/RConn1
  Switch/LConn1 -- E/RConn1 -- Diode/LConn1

== system ps_model/inverter/MOS based inverter/inverter/mosfet_3 ==
  Diode : fl_lib/Electrical/Electrical Elements/Diode  Vf=Vgamma V  Ron=Ron Ohm  Goff=1e-8 1/Ohm  i_specify=off  i_priority=None  i=0 A  i_nominal_specify=off  i_nominal_value=1  i_nominal_unit=A  v_specify=off  v_priority=None  v=0 V  v_nominal_specify=off  v_nominal_value=1  v_nominal_unit=V
  Switch : fl_lib/Electrical/Electrical Elements/Switch  R_closed=Ron Ohm  G_open=1e-8 1/Ohm  Threshold=7.5  i_specify=off  i_priority=None  i=0 A  i_nominal_specify=off  i_nominal_value=1  i_nominal_unit=A  v_specify=off  v_priority=None  v=0 V  v_nominal_specify=off  v_nominal_value=1  v_nominal_unit=V
  G : PMIOPort  Side=Left
  C : PMIOPort  Port=2  Side=Left
  E : PMIOPort  Port=3  Side=Right
  connections:
  Switch/RConn2 -- C/RConn1 -- Diode/RConn1
  Switch/RConn1 -- G/RConn1
  Switch/LConn1 -- E/RConn1 -- Diode/LConn1

== system ps_model/inverter/MOS based inverter/inverter/mosfet_4 ==
  Diode : fl_lib/Electrical/Electrical Elements/Diode  Vf=Vgamma V  Ron=Ron Ohm  Goff=1e-8 1/Ohm  i_specify=off  i_priority=None  i=0 A  i_nominal_specify=off  i_nominal_value=1  i_nominal_unit=A  v_specify=off  v_priority=None  v=0 V  v_nominal_specify=off  v_nominal_value=1  v_nominal_unit=V
  Switch : fl_lib/Electrical/Electrical Elements/Switch  R_closed=Ron Ohm  G_open=1e-8 1/Ohm  Threshold=7.5  i_specify=off  i_priority=None  i=0 A  i_nominal_specify=off  i_nominal_value=1  i_nominal_unit=A  v_specify=off  v_priority=None  v=0 V  v_nominal_specify=off  v_nominal_value=1  v_nominal_unit=V
  G : PMIOPort  Side=Left
  C : PMIOPort  Port=2  Side=Left
  E : PMIOPort  Port=3  Side=Right
  connections:
  Diode/LConn1 -- E/RConn1 -- Switch/LConn1
  Switch/RConn1 -- G/RConn1
  Diode/RConn1 -- C/RConn1 -- Switch/RConn2

== system ps_model/inverter/MOS based inverter/inverter/mosfet_5 ==
  Diode : fl_lib/Electrical/Electrical Elements/Diode  Vf=Vgamma V  Ron=Ron Ohm  Goff=1e-8 1/Ohm  i_specify=off  i_priority=None  i=0 A  i_nominal_specify=off  i_nominal_value=1  i_nominal_unit=A  v_specify=off  v_priority=None  v=0 V  v_nominal_specify=off  v_nominal_value=1  v_nominal_unit=V
  Switch : fl_lib/Electrical/Electrical Elements/Switch  R_closed=Ron Ohm  G_open=1e-8 1/Ohm  Threshold=7.5  i_specify=off  i_priority=None  i=0 A  i_nominal_specify=off  i_nominal_value=1  i_nominal_unit=A  v_specify=off  v_priority=None  v=0 V  v_nominal_specify=off  v_nominal_value=1  v_nominal_unit=V
  G : PMIOPort  Side=Left
  C : PMIOPort  Port=2  Side=Left
  E : PMIOPort  Port=3  Side=Right
  connections:
  Switch/RConn2 -- C/RConn1 -- Diode/RConn1
  Switch/RConn1 -- G/RConn1
  Switch/LConn1 -- E/RConn1 -- Diode/LConn1

== system ps_model/inverter/MOS based inverter/inverter/mosfet_6 ==
  Diode : fl_lib/Electrical/Electrical Elements/Diode  Vf=Vgamma V  Ron=Ron Ohm  Goff=1e-8 1/Ohm  i_specify=off  i_priority=None  i=0 A  i_nominal_specify=off  i_nominal_value=1  i_nominal_unit=A  v_specify=off  v_priority=None  v=0 V  v_nominal_specify=off  v_nominal_value=1  v_nominal_unit=V
  Switch : fl_lib/Electrical/Electrical Elements/Switch  R_closed=Ron Ohm  G_open=1e-8 1/Ohm  Threshold=7.5  i_specify=off  i_priority=None  i=0 A  i_nominal_specify=off  i_nominal_value=1  i_nominal_unit=A  v_specify=off  v_priority=None  v=0 V  v_nominal_specify=off  v_nominal_value=1  v_nominal_unit=V
  G : PMIOPort  Side=Left
  C : PMIOPort  Port=2  Side=Left
  E : PMIOPort  Port=3  Side=Right
  connections:
  Diode/LConn1 -- E/RConn1 -- Switch/LConn1
  Switch/RConn1 -- G/RConn1
  Diode/RConn1 -- C/RConn1 -- Switch/RConn2

== system ps_model/inverter/MOS based inverter/spwm/modulator1 ==
  u : Inport
  v : Inport  Port=2
  w : Inport  Port=3
  phase : Inport  Port=4
  Bus Creator3 : BusCreator  Inputs=6
  PWM generator 1 : Subsystem  mask{f=fPWM_INV, m_up=1, m_low=0, dead_time=0, pos_cmd_gate=15, neg_cmd_gate=-10, polarity=1}
      mask prompts: f "Frequency (Hz)"; m_up "Max Input Modulation Value"; m_low "Min Input Modulation Value"; dead_time "Dead Time (s)"; pos_cmd_gate "Positive Gate Voltage (V)"; neg_cmd_gate "Negative Gate Voltage (V)"; polarity "Polarity (pu)"
  PWM generator 2 : Subsystem  mask{f=fPWM_INV, m_up=1, m_low=0, dead_time=0, pos_cmd_gate=15, neg_cmd_gate=-10, polarity=1}
      mask prompts: f "Frequency (Hz)"; m_up "Max Input Modulation Value"; m_low "Min Input Modulation Value"; dead_time "Dead Time (s)"; pos_cmd_gate "Positive Gate Voltage (V)"; neg_cmd_gate "Negative Gate Voltage (V)"; polarity "Polarity (pu)"
  PWM generator 3 : Subsystem  mask{f=fPWM_INV, m_up=1, m_low=0, dead_time=0, pos_cmd_gate=15, neg_cmd_gate=-10, polarity=1}
      mask prompts: f "Frequency (Hz)"; m_up "Max Input Modulation Value"; m_low "Min Input Modulation Value"; dead_time "Dead Time (s)"; pos_cmd_gate "Positive Gate Voltage (V)"; neg_cmd_gate "Negative Gate Voltage (V)"; polarity "Polarity (pu)"
  cmd_gates : Outport
  wires:
  Bus Creator3/1 -> cmd_gates/1
  PWM generator 1/1(m1) -> Bus Creator3/1  "gate_cmd_Q1"
  PWM generator 3/2(m2) -> Bus Creator3/6  "gate_cmd_Q6"
  PWM generator 2/2(m2) -> Bus Creator3/4  "gate_cmd_Q4"
  PWM generator 2/1(m1) -> Bus Creator3/3  "gate_cmd_Q3"
  PWM generator 3/1(m1) -> Bus Creator3/5  "gate_cmd_Q5"
  PWM generator 1/2(m2) -> Bus Creator3/2  "gate_cmd_Q2"
  phase/1 -> PWM generator 1/2(phase), PWM generator 2/2(phase), PWM generator 3/2(phase)
  v/1 -> PWM generator 2/1(m_index)
  w/1 -> PWM generator 3/1(m_index)
  u/1 -> PWM generator 1/1(m_index)

== system ps_model/inverter/MOS based inverter/sv_pwm/modulator1 ==
  u : Inport
  v : Inport  Port=2
  w : Inport  Port=3
  phase : Inport  Port=4
  Bus Creator3 : BusCreator  Inputs=6
  PWM generator 1 : Subsystem  mask{f=fPWM_INV, m_up=1, m_low=0, dead_time=0, pos_cmd_gate=15, neg_cmd_gate=-10, polarity=1}
      mask prompts: f "Frequency (Hz)"; m_up "Max Input Modulation Value"; m_low "Min Input Modulation Value"; dead_time "Dead Time (s)"; pos_cmd_gate "Positive Gate Voltage (V)"; neg_cmd_gate "Negative Gate Voltage (V)"; polarity "Polarity (pu)"
  PWM generator 2 : Subsystem  mask{f=fPWM_INV, m_up=1, m_low=0, dead_time=0, pos_cmd_gate=15, neg_cmd_gate=-10, polarity=1}
      mask prompts: f "Frequency (Hz)"; m_up "Max Input Modulation Value"; m_low "Min Input Modulation Value"; dead_time "Dead Time (s)"; pos_cmd_gate "Positive Gate Voltage (V)"; neg_cmd_gate "Negative Gate Voltage (V)"; polarity "Polarity (pu)"
  PWM generator 3 : Subsystem  mask{f=fPWM_INV, m_up=1, m_low=0, dead_time=0, pos_cmd_gate=15, neg_cmd_gate=-10, polarity=1}
      mask prompts: f "Frequency (Hz)"; m_up "Max Input Modulation Value"; m_low "Min Input Modulation Value"; dead_time "Dead Time (s)"; pos_cmd_gate "Positive Gate Voltage (V)"; neg_cmd_gate "Negative Gate Voltage (V)"; polarity "Polarity (pu)"
  cmd_gates : Outport
  wires:
  u/1 -> PWM generator 1/1(m_index)
  w/1 -> PWM generator 3/1(m_index)
  v/1 -> PWM generator 2/1(m_index)
  phase/1 -> PWM generator 3/2(phase), PWM generator 2/2(phase), PWM generator 1/2(phase)
  PWM generator 1/2(m2) -> Bus Creator3/2  "gate_cmd_Q2"
  PWM generator 3/1(m1) -> Bus Creator3/5  "gate_cmd_Q5"
  PWM generator 2/1(m1) -> Bus Creator3/3  "gate_cmd_Q3"
  PWM generator 2/2(m2) -> Bus Creator3/4  "gate_cmd_Q4"
  PWM generator 3/2(m2) -> Bus Creator3/6  "gate_cmd_Q6"
  PWM generator 1/1(m1) -> Bus Creator3/1  "gate_cmd_Q1"
  Bus Creator3/1 -> cmd_gates/1

== system ps_model/inverter/instantaneus_power/abc2alphabeta/abc2alphabeta ==
  a : Inport
  b : Inport  Port=2
  c : Inport  Port=3
  Gain1 : Gain  Gain=-1/2
  Gain11 : Gain  Gain=-1/2
  Gain2 : Gain  Gain=0
  Gain3 : Gain  Gain=sqrt(3)/2
  Gain4 : Gain  Gain=-sqrt(3)/2
  Gain8 : Gain  Gain=2/3
  Gain9 : Gain  Gain=2/3
  Sum : Sum  Inputs=+++
  Sum1 : Sum  Inputs=+++
  "alpha " : Outport  VectorParamsAs1DForOutWhenUnconnected=off
  "beta " : Outport  Port=2  VectorParamsAs1DForOutWhenUnconnected=off
  wires:
  Gain11/1 -> Sum/2
  Gain1/1 -> Sum/3
  Gain9/1 -> "beta "/1
  Gain8/1 -> "alpha "/1
  Gain2/1 -> Sum1/1
  Gain3/1 -> Sum1/2
  Gain4/1 -> Sum1/3
  a/1 -> Gain2/1, Sum/1
  c/1 -> Gain4/1, Gain1/1
  b/1 -> Gain3/1, Gain11/1
  Sum/1 -> Gain8/1
  Sum1/1 -> Gain9/1

== system ps_model/inverter/instantaneus_power/abc2alphabeta /abc->alphabeta ==
  a : Inport
  b : Inport  Port=2
  c : Inport  Port=3
  Gain1 : Gain  Gain=-1/2
  Gain11 : Gain  Gain=-1/2
  Gain2 : Gain  Gain=0
  Gain3 : Gain  Gain=sqrt(3)/2
  Gain4 : Gain  Gain=-sqrt(3)/2
  Gain8 : Gain  Gain=2/3
  Gain9 : Gain  Gain=2/3
  Sum : Sum  Inputs=+++
  Sum1 : Sum  Inputs=+++
  "alpha " : Outport  VectorParamsAs1DForOutWhenUnconnected=off
  "beta " : Outport  Port=2  VectorParamsAs1DForOutWhenUnconnected=off
  wires:
  Sum1/1 -> Gain9/1
  Sum/1 -> Gain8/1
  b/1 -> Gain11/1, Gain3/1
  c/1 -> Gain1/1, Gain4/1
  a/1 -> Sum/1, Gain2/1
  Gain4/1 -> Sum1/3
  Gain3/1 -> Sum1/2
  Gain2/1 -> Sum1/1
  Gain8/1 -> "alpha "/1
  Gain9/1 -> "beta "/1
  Gain1/1 -> Sum/3
  Gain11/1 -> Sum/2

== system ps_model/rectifier/rectifier/dclink_measure/R_derating ==
  Step : Step  After=107.4e3/2  SampleTime=0
  Step1 : Step  Time=1.1  After=-107.4e3/2  SampleTime=0
  Sum : Sum  Inputs=|++
  DR : Outport
  wires:
  Step1/1 -> Sum/2
  Step/1 -> Sum/1
  Sum/1 -> DR/1

== system ps_model/battery_system/battery_system/LithiumIonBattery/SOC_estimator/Kalman_observer ==
  vout(k) : Inport
  Constant : Constant  Value=tsample
  Constant1 : Constant  Value=Q
  Constant2 : Constant  Value=q1Kalman
  Constant3 : Constant  Value=q2Kalman
  Constant4 : Constant  Value=q3Kalman
  Constant5 : Constant  Value=rKalman
  Constant6 : Constant  Value=tsample
  Constant7 : Constant  Value=Q
  Selector : Selector  InputPortWidth=3  IndexOptions=Index vector (dialog)  Indices=1  OutputSizes=1
  Unit Delay4 : UnitDelay  SampleTime=tsample  HasFrameUpgradeWarning=on
  kalman_observer_gains : MATLAB Function  TreatAsAtomicUnit=on  SystemSampleTime=tsample
  lithium-ion battery model : MATLAB Function  TreatAsAtomicUnit=on  SystemSampleTime=tsample
  vout/vout_hat : Scope  Commented=on  NumInputPorts=2
      settings: SampleTime=tsample  ActiveDisplayYMinimum=-781.71351  ActiveDisplayYMaximum=896.62262
  x(k+1|k) : Outport
  SOC : Outport  Port=2
  wires:
  lithium-ion battery model/2(u) -> vout/vout_hat/2  "vout_hat"
  vout(k)/1 -> lithium-ion battery model/7(vout), vout/vout_hat/1
  lithium-ion battery model/3(x) -> x(k+1|k)/1, Selector/1  "x(k+1|k)"
  kalman_observer_gains/2(l2) -> lithium-ion battery model/5(l2)
  Constant6/1 -> kalman_observer_gains/2(ts)
  lithium-ion battery model/1(SOC) -> SOC/1  "SOC"
  Constant7/1 -> kalman_observer_gains/8(Q)
  kalman_observer_gains/3(l3) -> lithium-ion battery model/6(l3)
  Constant1/1 -> lithium-ion battery model/3(Q)
  Constant5/1 -> kalman_observer_gains/7(r)
  [im] -> kalman_observer_gains/1(i)
  Constant4/1 -> kalman_observer_gains/6(q3)
  Constant2/1 -> kalman_observer_gains/4(q1)
  kalman_observer_gains/1(l1) -> lithium-ion battery model/4(l1)
  Constant/1 -> lithium-ion battery model/2(ts)
  Constant3/1 -> kalman_observer_gains/5(q2)
  Unit Delay4/1 -> kalman_observer_gains/3(z)  "x(k|k-1)"
  Selector/1 -> Unit Delay4/1
  [im] -> lithium-ion battery model/1(i)

== system ps_model/battery_system/battery_system/LithiumIonBattery/lithium ion cell analytical ocv/white_noise ==
  in : Inport
  Band-Limited White Noise : simulink/Sources/Band-Limited White Noise  Commented=on  Cov=tsample  Ts=tsample  seed=[23341]
  Sum2 : Sum  Inputs=|++
  out : Outport
  wires:
  Band-Limited White Noise/1 -> Sum2/2
  Sum2/1 -> out/1
  in/1 -> Sum2/1

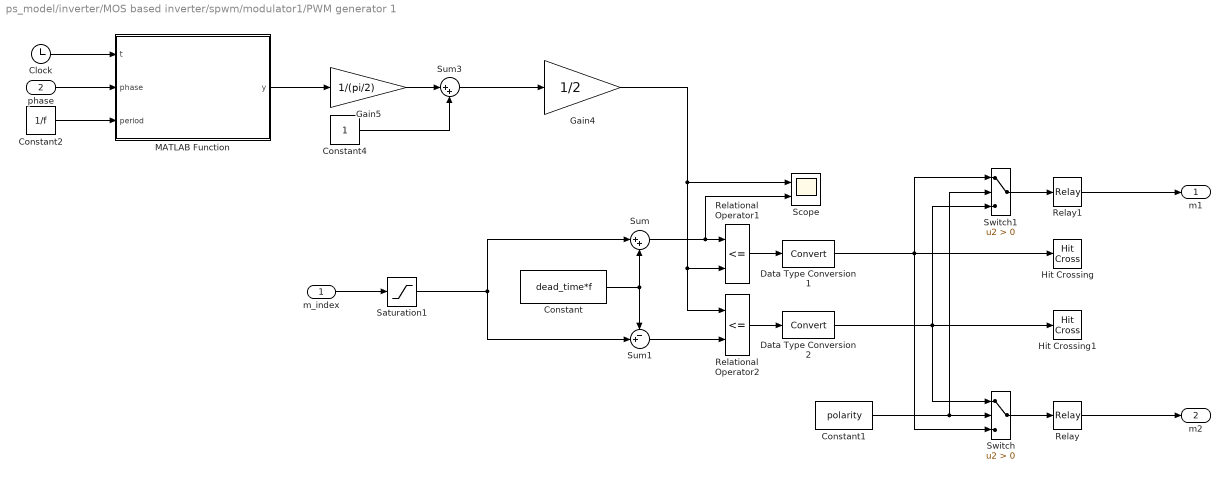
== system ps_model/inverter/MOS based inverter/spwm/modulator1/PWM generator 1 ==
  m_index : Inport
  phase : Inport  Port=2
  Clock : Clock
  Constant : Constant  Value=dead_time*f
  Constant1 : Constant  Value=polarity
  Constant2 : Constant  Value=1/f
  Constant4 : Constant
  Data Type Conversion1 : DataTypeConversion
  Data Type Conversion2 : DataTypeConversion
  Gain4 : Gain  Gain=1/2
  Gain5 : Gain  Gain=1/(pi/2)
  Hit Crossing : HitCross  ShowOutputPort=off
  Hit Crossing1 : HitCross  ShowOutputPort=off
  MATLAB Function : MATLAB Function  TreatAsAtomicUnit=on
  Relational Operator1 : RelationalOperator  Operator=<=  InputSameDT=off
  Relational Operator2 : RelationalOperator  Operator=<=  InputSameDT=off
  Relay : Relay  OnOutputValue=pos_cmd_gate  OffOutputValue=neg_cmd_gate
  Relay1 : Relay  OnOutputValue=pos_cmd_gate  OffOutputValue=neg_cmd_gate
  Saturation1 : Saturate  UpperLimit=m_up  LowerLimit=m_low
  Scope : Scope  NumInputPorts=2
      settings: ActiveDisplayYMinimum=-0.125  ActiveDisplayYMaximum=1.125
  Sum : Sum  Inputs=|++  SaturateOnIntegerOverflow=on
  Sum1 : Sum  Inputs=-+|  SaturateOnIntegerOverflow=on
  Sum3 : Sum  Inputs=|++
  Switch : Switch  Criteria=u2 > Threshold  SaturateOnIntegerOverflow=off  InputSameDT=off
  Switch1 : Switch  Criteria=u2 > Threshold  SaturateOnIntegerOverflow=off  InputSameDT=off
  m1 : Outport
  m2 : Outport  Port=2
  wires:
  Relay1/1 -> m1/1
  Switch1/1 -> Relay1/1
  Constant1/1 -> Switch/2, Switch1/2
  Relay/1 -> m2/1
  Constant4/1 -> Sum3/2
  Sum3/1 -> Gain4/1
  Gain5/1 -> Sum3/1
  MATLAB Function/1(y) -> Gain5/1
  phase/1 -> MATLAB Function/2(phase)
  Constant2/1 -> MATLAB Function/3(period)
  Clock/1 -> MATLAB Function/1(t)
  Switch/1 -> Relay/1
  Data Type Conversion1/1 -> Switch1/1, Switch/3, Hit Crossing/1
  Gain4/1 -> Scope/1, Relational Operator1/2, Relational Operator2/1
  Sum1/1 -> Relational Operator2/2
  Sum/1 -> Scope/2, Relational Operator1/1
  Saturation1/1 -> Sum1/2, Sum/1
  Constant/1 -> Sum1/1, Sum/2
  Data Type Conversion2/1 -> Hit Crossing1/1, Switch1/3, Switch/1
  Relational Operator2/1 -> Data Type Conversion2/1
  m_index/1 -> Saturation1/1
  Relational Operator1/1 -> Data Type Conversion1/1

== system ps_model/inverter/MOS based inverter/spwm/modulator1/PWM generator 2 ==
  m_index : Inport
  phase : Inport  Port=2
  Clock : Clock
  Constant : Constant  Value=dead_time*f
  Constant1 : Constant  Value=polarity
  Constant2 : Constant  Value=1/f
  Constant4 : Constant
  Data Type Conversion1 : DataTypeConversion
  Data Type Conversion2 : DataTypeConversion
  Gain4 : Gain  Gain=1/2
  Gain5 : Gain  Gain=1/(pi/2)
  Hit Crossing : HitCross  ShowOutputPort=off
  Hit Crossing1 : HitCross  ShowOutputPort=off
  MATLAB Function : MATLAB Function  TreatAsAtomicUnit=on
  Relational Operator1 : RelationalOperator  Operator=<=  InputSameDT=off
  Relational Operator2 : RelationalOperator  Operator=<=  InputSameDT=off
  Relay : Relay  OnOutputValue=pos_cmd_gate  OffOutputValue=neg_cmd_gate
  Relay1 : Relay  OnOutputValue=pos_cmd_gate  OffOutputValue=neg_cmd_gate
  Saturation1 : Saturate  UpperLimit=m_up  LowerLimit=m_low
  Sum : Sum  Inputs=|++  SaturateOnIntegerOverflow=on
  Sum1 : Sum  Inputs=-+|  SaturateOnIntegerOverflow=on
  Sum3 : Sum  Inputs=|++
  Switch : Switch  Criteria=u2 > Threshold  SaturateOnIntegerOverflow=off  InputSameDT=off
  Switch1 : Switch  Criteria=u2 > Threshold  SaturateOnIntegerOverflow=off  InputSameDT=off
  m1 : Outport
  m2 : Outport  Port=2
  wires:
  Relational Operator1/1 -> Data Type Conversion1/1
  m_index/1 -> Saturation1/1
  Relational Operator2/1 -> Data Type Conversion2/1
  Data Type Conversion2/1 -> Switch/1, Switch1/3, Hit Crossing1/1
  Constant/1 -> Sum/2, Sum1/1
  Saturation1/1 -> Sum/1, Sum1/2
  Sum/1 -> Relational Operator1/1
  Sum1/1 -> Relational Operator2/2
  Gain4/1 -> Relational Operator2/1, Relational Operator1/2
  Data Type Conversion1/1 -> Hit Crossing/1, Switch/3, Switch1/1
  Switch/1 -> Relay/1
  Clock/1 -> MATLAB Function/1(t)
  Constant2/1 -> MATLAB Function/3(period)
  phase/1 -> MATLAB Function/2(phase)
  MATLAB Function/1(y) -> Gain5/1
  Gain5/1 -> Sum3/1
  Sum3/1 -> Gain4/1
  Constant4/1 -> Sum3/2
  Relay/1 -> m2/1
  Constant1/1 -> Switch1/2, Switch/2
  Switch1/1 -> Relay1/1
  Relay1/1 -> m1/1
